simulink model "test_canards_sim"  (R2026b)
settings: Solver=VariableStepAuto  StopTime=25
values from neighbouring files (symbols this model uses):
  Area = 0.014    [Full_Rocket_Constants.m]    (also in TestRocketSetup.m = 0.00817128249199)
  BF_H = 0.14    [Full_Rocket_Constants.m]    (also in TestRocketSetup.m = 0.102)
  BF_NFins = 4    [Full_Rocket_Constants.m]    (also in TestRocketSetup.m)
  BF_plan = ((BF_TC+BF_RC)/2)*BF_H    (= 0.0329)    [Full_Rocket_Constants.m]    (also in TestRocketSetup.m = 0.0162129)
  BF_SA = deg2rad(58.3)    [Full_Rocket_Constants.m]    (also in TestRocketSetup.m = atan(BF_SL/BF_H))
  BF_t = 0.003    [TestRocketSetup.m]
  BF_X = 7.00    (= 7)    [Full_Rocket_Constants.m]    (also in TestRocketSetup.m = 1.626)
  BF_yMac = (BF_H/3)*((BF_RC+(2*BF_TC))/(BF_RC+BF_TC))    (= 0.0617588652482)    [Full_Rocket_Constants.m]    (also in TestRocketSetup.m = 0.0435080213904)
  boost_end = boosterCurve(length(boosterCurve), 1)    [Full_Rocket_Constants.m]    (also in TestRocketSetup.m)
  boost_start = boosterCurve(1, 1)    [Full_Rocket_Constants.m]    (also in TestRocketSetup.m)
  boost_t_cg = boost_data(:,1)    [Full_Rocket_Constants.m]    (also in TestRocketSetup.m)
  boost_x_cg = boost_data(:,3)    [Full_Rocket_Constants.m]    (also in TestRocketSetup.m = boost_data(:,3)/100)
  Booster_Length = 4.73    [Full_Rocket_Constants.m]    (also in TestRocketSetup.m = 1.92)
  Booster_MotorDiam = 0.098    [Full_Rocket_Constants.m]    (also in TestRocketSetup.m = 0.075)
  boosterCurve = thrustCurve("Data/Cesaroni_2856L910-P.csv")    [TestRocketSetup.m]
  boosterISP = 223    [Full_Rocket_Constants.m]    (also in TestRocketSetup.m = 229)
  cbar_BF = (2/3)*(BF_RC^2 + BF_RC*BF_TC + BF_TC^2)/(BF_RC + BF_TC)    (= 0.244771631206)    [Full_Rocket_Constants.m]    (also in TestRocketSetup.m = 0.169240452973)
  cbar_CR = CR_Plan/CR_Span    [Full_Rocket_Constants.m]    (also in TestRocketSetup.m = 0.0169333333333)
  CR_LE = atan(CR_SL/CR_Span)    [TestRocketSetup.m]
  CR_mC = 0    [Full_Rocket_Constants.m]    (also in TestRocketSetup.m = atan((CR_SL + CR_TC/2 - CR_RC/2)/CR_Span))
  CR_Plan = 0    [Full_Rocket_Constants.m]    (also in TestRocketSetup.m = 0.000381)
  CR_pos = 0    [Full_Rocket_Constants.m]    (also in TestRocketSetup.m = 0.495166666667)
  CR_Span = sqrt(CR_AR*CR_Plan)    [Full_Rocket_Constants.m]    (also in TestRocketSetup.m = 0.03)
  CR_t = 0.003    [TestRocketSetup.m]
  CR_yMAC = (CR_Span/3)*(CR_RC + 2*CR_TC)/(CR_RC + CR_TC)    (= 0.01)    [TestRocketSetup.m]
  Diam = 0.157    [Full_Rocket_Constants.m]    (also in TestRocketSetup.m = 0.102)
  Gc_BF = atan((BF_SL + BF_TC/2 - BF_RC/2)/BF_H)    [Full_Rocket_Constants.m]    (also in TestRocketSetup.m)
  Ixx_empty = 0.016109    [TestRocketSetup.m]
  Ixx_full = 0.017068    [TestRocketSetup.m]
  Iyy_empty = 3.018769    [TestRocketSetup.m]
  Iyy_full = 3.518905    [TestRocketSetup.m]
  NC_aBase = pi*(NC_dBase/2)^2    (= 0.0134782178821)    [Full_Rocket_Constants.m]    (also in TestRocketSetup.m = 0.00817128249199)
  NC_aPlan = 0.03355206    [Full_Rocket_Constants.m]    (also in TestRocketSetup.m = integral(@(x) 2*NC_rx(x), 0, NC_L))
  NC_aTop = pi*(NC_dTop/2)^2    (= 0)    [Full_Rocket_Constants.m]    (also in TestRocketSetup.m = 7.85398163397e-19)
  NC_CP = NC_L*0.466    (= 0.177546)    [Full_Rocket_Constants.m]    (also in TestRocketSetup.m = 0.189196)
  NC_dBase = 0.131    [Full_Rocket_Constants.m]    (also in TestRocketSetup.m = 0.102)
  NC_kappa = 1    [TestRocketSetup.m]
  NC_L = 0.381    [Full_Rocket_Constants.m]    (also in TestRocketSetup.m = 0.406)
  NC_phiJoint = 0    [TestRocketSetup.m]
  NC_Xlift = NC_Xlift_numerator / NC_aPlan    [Full_Rocket_Constants.m]    (also in TestRocketSetup.m)
  SC_L =     [Full_Rocket_Constants.m]    (also in TestRocketSetup.m = 0.229)
  spincan_radius = 0.0889    [Full_Rocket_Constants.m]    (also in TestRocketSetup.m = 0.0635)
  SurfaceRoughness = 60e-6    (= 6e-05)    [Full_Rocket_Constants.m]    (also in TestRocketSetup.m)
  TR_L =     [Full_Rocket_Constants.m]    (also in TestRocketSetup.m = 0.102)
  xMAC_BF = (BF_SL/3)*(BF_RC + 2*BF_TC)/(BF_RC + BF_TC)    (= 0.100137588652)    [Full_Rocket_Constants.m]    (also in TestRocketSetup.m = 0.0789116074237)
libraries: simulink x4, slpidlib x2, sl_discontinuities x2, aerolibwind2 x2, aerolibanim x1, aerolibatmos2 x1, aerolibasang x1
settings Model: SimulationMode=accelerator  Creator=linda  LastModifiedBy=linda
settings RTWCC: GPUComputeCapability=5.0

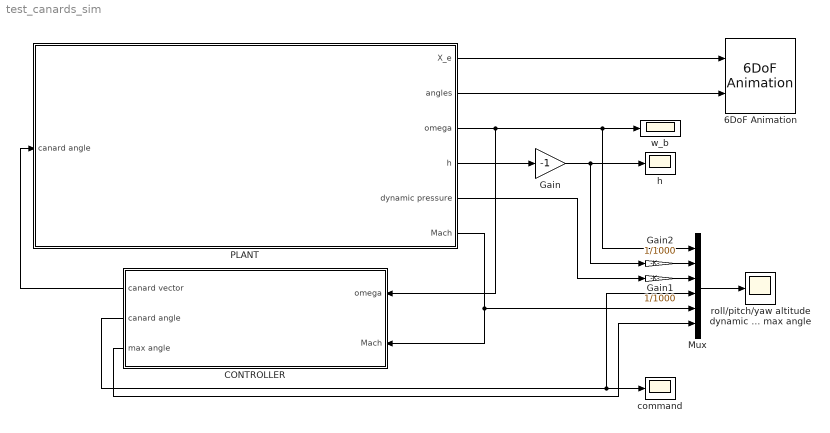
== system test_canards_sim ==
  6DoF Animation : aerolibanim/6DoF Animation  u1=[-1000 1000 -1000 1000 -2500 100]  u2=0.1  u3=250  u4=[1e6 1e6 1e6]  u5=Fixed position  u6=[3000 -3200 -1200]  u7=35  u8=on
  CONTROLLER : Subsystem
      settings: PortSchema="{\"entries\":[{\"content\":{\"sides\":[{\"content\":{\"connectorIds\":[\"Out1\",\"Out2\",\"Out3\"]},\"type\":\"ConnectorPlacement.EquallySpacedRectSide\",\"uuid\":\"acb4eb02-5623-4936-ab90-b0a31d594ccc\"},{\"content\":{\"connectorIds\":[\"In1\",\"In2\"],\"side\":\"RIGHT\"},\"type\":\"ConnectorPlacement.EquallySpacedRectSide\",\"uuid\":\"32f7e7ec-6d55-4d58-a621-02218861ecad\"},{\"content\":{\"side\":\"TOP\"},\"type\":\"ConnectorPlacement.EquallySpacedRectSide\",\"uuid\":\"63922e56-f870-4494-8f72-8c2e527eb7e4\"}]},\"type\":\"ConnectorPlacement.EquallySpacedConnector\",\"uuid\":\"1a722234-757d-46dd-a7b9-af51da458303\"}],\"packageUris\":[\"http://schema.mathworks.com/mf0/Connector/R2020b\"],\"version\":\"1.0\"}"
  Gain : Gain  Gain=-1
  Gain1 : Gain  Gain=1/1000
  Gain2 : Gain  Gain=1/1000
  Mux : Mux  Inputs=6
  PLANT : Subsystem
  command : Scope
      settings: ActiveDisplayYMinimum=-0.098392544287147957  ActiveDisplayYMaximum=0.020869012493307838  DataLoggingVariableName=ScopeData3
  h : Scope
      settings: ActiveDisplayYMinimum=1452.8796933312713  ActiveDisplayYMaximum=2766.4256793789323  DataLoggingVariableName=ScopeData2
  roll/pitch/yaw altitude dynamic pressure command mach max angle : Scope
      settings: ActiveDisplayYMinimum=-0.92690613477267036  ActiveDisplayYMaximum=0.910025444475978  DataLoggingVariableName=ScopeData4
  w_b : Scope
      settings: ActiveDisplayYMinimum=-3.5754328935781414  ActiveDisplayYMaximum=12.108972824331008
  wires:
  CONTROLLER/1(canard vector) -> PLANT/1(canard angle)
  PLANT/1(X_e) -> 6DoF Animation/1
  PLANT/2(angles) -> 6DoF Animation/2
  PLANT/3(omega) -> Mux/1, w_b/1, CONTROLLER/1(omega)
  PLANT/4(h) -> Gain/1
  Gain/1 -> Gain2/1, h/1
  CONTROLLER/2(canard angle) -> command/1, Mux/4
  Mux/1 -> roll/pitch/yaw altitude dynamic pressure command mach max angle/1
  Gain1/1 -> Mux/3
  PLANT/5(dynamic pressure) -> Gain1/1
  Gain2/1 -> Mux/2
  PLANT/6(Mach) -> CONTROLLER/2(Mach), Mux/5
  CONTROLLER/3(max angle) -> Mux/6

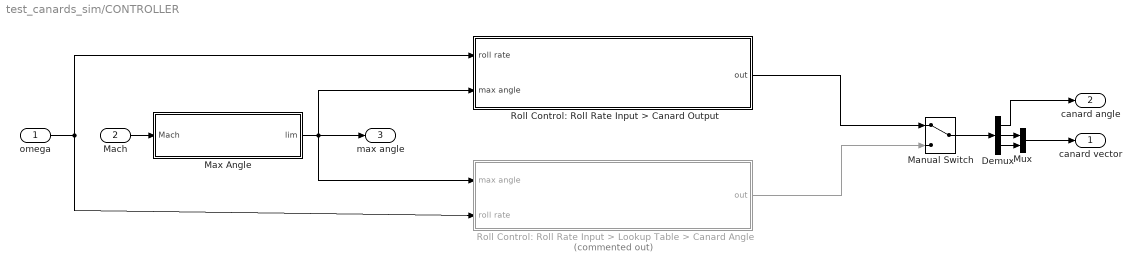
== system test_canards_sim/CONTROLLER ==
  omega : Inport
  Mach : Inport  Port=2
  Demux : Demux  Outputs=3
  Manual Switch : ManualSwitch
  Max Angle : Subsystem
  Mux : Mux  Inputs=2
  Roll Control: Roll Rate Input > Canard Output : Subsystem
  Roll Control: Roll Rate Input > Lookup Table > Canard Angle : Subsystem  Commented=on
  canard vector : Outport
  canard angle : Outport  Port=2
  max angle : Outport  Port=3
  wires:
  omega/1 -> Roll Control: Roll Rate Input > Canard Output/1(roll rate), Roll Control: Roll Rate Input > Lookup Table > Canard Angle/2(roll rate)
  Mach/1 -> Max Angle/1(Mach)
  Max Angle/1(lim) -> Roll Control: Roll Rate Input > Lookup Table > Canard Angle/1(max angle), Roll Control: Roll Rate Input > Canard Output/2(max angle), max angle/1
  Roll Control: Roll Rate Input > Canard Output/1(out) -> Manual Switch/1
  Manual Switch/1 -> Demux/1
  Demux/1 -> canard angle/1
  Roll Control: Roll Rate Input > Lookup Table > Canard Angle/1(out) -> Manual Switch/2
  Demux/2 -> Mux/1
  Demux/3 -> Mux/2
  Mux/1 -> canard vector/1

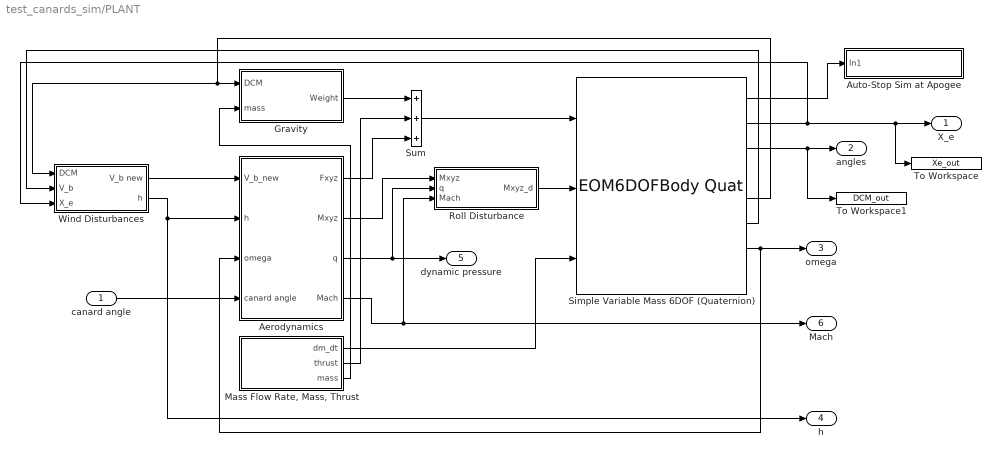
== system test_canards_sim/PLANT ==
  canard angle : Inport
  Aerodynamics : Subsystem
  Auto-Stop Sim at Apogee : Subsystem
  Gravity : Subsystem
  "Mass Flow Rate, Mass, Thrust" : Subsystem
  Roll Disturbance : Subsystem
  Simple Variable Mass 6DOF (Quaternion) : EOM6DOFBodyQuat  mtype=Simple Variable  eul_0=[0 deg2rad(85) 0]  mass_0=BoosterWetMass  mass_e=BoosterBurnoutMass  mass_f=BoosterWetMass  inertia_e=diag([Ixx_empty, Iyy_empty, Iyy_empty])  inertia_f=diag([Ixx_full, Iyy_full, Iyy_full])
  Sum : Sum  Inputs=+++
  To Workspace : ToWorkspace  VariableName=Xe_out  SaveFormat=Timeseries  SampleTime=-1
  To Workspace1 : ToWorkspace  VariableName=DCM_out  SaveFormat=Timeseries  SampleTime=-1
  Wind Disturbances : Subsystem
  X_e : Outport
  angles : Outport  Port=2
  omega : Outport  Port=3
  h : Outport  Port=4
  dynamic pressure : Outport  Port=5
  Mach : Outport  Port=6
  wires:
  Wind Disturbances/2(h) -> h/1, Aerodynamics/2(h)
  Simple Variable Mass 6DOF (Quaternion)/7 -> omega/1, Aerodynamics/3(omega)
  Simple Variable Mass 6DOF (Quaternion)/2 -> To Workspace/1, X_e/1, Wind Disturbances/3(X_e)
  Sum/1 -> Simple Variable Mass 6DOF (Quaternion)/1
  Gravity/1(Weight) -> Sum/1
  Aerodynamics/1(Fxyz) -> Sum/3
  Simple Variable Mass 6DOF (Quaternion)/5 -> Wind Disturbances/1(DCM), Gravity/1(DCM)
  Wind Disturbances/1(V_b new) -> Aerodynamics/1(V_b_new)
  Simple Variable Mass 6DOF (Quaternion)/6 -> Wind Disturbances/2(V_b)
  "Mass Flow Rate, Mass, Thrust"/1(dm_dt) -> Simple Variable Mass 6DOF (Quaternion)/3
  "Mass Flow Rate, Mass, Thrust"/2(thrust) -> Sum/2
  "Mass Flow Rate, Mass, Thrust"/3(mass) -> Gravity/2(mass)
  Simple Variable Mass 6DOF (Quaternion)/1 -> Auto-Stop Sim at Apogee/1(In1)
  Simple Variable Mass 6DOF (Quaternion)/3 -> To Workspace1/1, angles/1
  canard angle/1 -> Aerodynamics/4(canard angle)
  Aerodynamics/2(Mxyz) -> Roll Disturbance/1(Mxyz)
  Roll Disturbance/1(Mxyz_d) -> Simple Variable Mass 6DOF (Quaternion)/2
  Aerodynamics/3(q) -> dynamic pressure/1, Roll Disturbance/2(q)
  Aerodynamics/4(Mach) -> Roll Disturbance/3(Mach), Mach/1

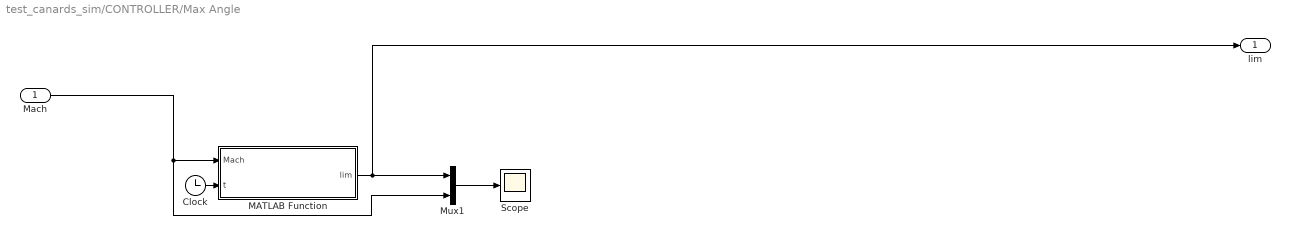
== system test_canards_sim/CONTROLLER/Max Angle ==
  Mach : Inport
  Clock : Clock
  MATLAB Function : MATLAB Function  TreatAsAtomicUnit=on
  Mux1 : Mux  Inputs=2
  Scope : Scope
      settings: ActiveDisplayYMinimum=-0.10058311536277464  ActiveDisplayYMaximum=0.91689608071086814  DataLoggingVariableName=ScopeData8
  lim : Outport
  wires:
  Clock/1 -> MATLAB Function/2(t)
  Mach/1 -> MATLAB Function/1(Mach), Mux1/2
  MATLAB Function/1(lim) -> lim/1, Mux1/1
  Mux1/1 -> Scope/1

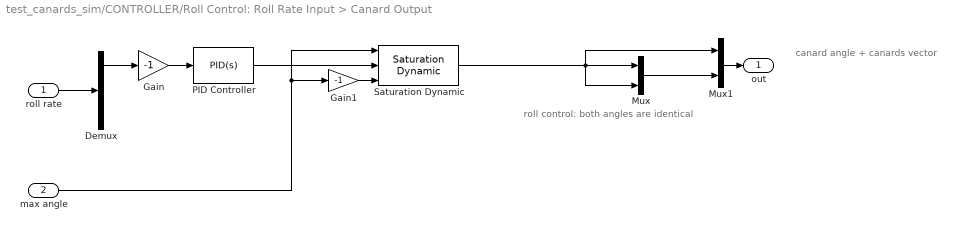
== system test_canards_sim/CONTROLLER/Roll Control: Roll Rate Input > Canard Output ==
  note: canard angle
      | +
      | canards vector
  note: roll control: both angles are identical
  roll rate : Inport
  max angle : Inport  Port=2
  Demux : Demux  Outputs=3
  Gain : Gain  Gain=-1
  Gain1 : Gain  Gain=-1
  Mux : Mux  Inputs=2
  Mux1 : Mux  Inputs=2
  PID Controller : slpidlib/PID Controller  Controller=PID  Form=Parallel  TimeDomain=Continuous-time  UseExternalTs=off  SampleTime=-1  IntegratorMethod=Forward Euler  FilterMethod=Forward Euler  ControllerParametersSource=internal  P=2.1  I=0.75  UseKiTs=off  D=0.2  UseExternalDerivativeSource=off  N=100  UseFilter=on  TunerSelectOption=Transfer Function Based (PID Tuner App)  InitialConditionSource=internal  InitialConditionForIntegrator=0  InitialConditionForFilter=0  DifferentiatorICPrevScaledInput=0  ExternalReset=none  TrackingMode=off  Kt=1  LimitOutput=off  SatLimitsSource=internal  UpperSaturationLimit=deg2rad(15)  LowerSaturationLimit=deg2rad(-15)  LinearizeAsGain=on  AntiWindupMode=clamping  Kb=1  LimitIntegrator=off  UpperIntegratorSaturationLimit=inf  LowerIntegratorSaturationLimit=-inf  POutMin=[]  POutMax=[]  IOutMin=[]  IOutMax=[]  DOutMin=[]  DOutMax=[]  NOutMin=[]  NOutMax=[]  SumOutMin=[]  SumOutMax=[]  SaturationOutMin=[]  SaturationOutMax=[]  PParamMin=[]  PParamMax=[]  IParamMin=[]  IParamMax=[]  DParamMin=[]  DParamMax=[]  NParamMin=[]  NParamMax=[]  KbParamMin=[]  KbParamMax=[]  KtParamMin=[]  KtParamMax=[]  KbOutMin=[]  KbOutMax=[]  KtOutMin=[]  KtOutMax=[]  IntegratorOutMin=[]  IntegratorOutMax=[]  FilterOutMin=[]  FilterOutMax=[]  SumI1OutMin=[]  SumI1OutMax=[]  SumI2OutMin=[]  SumI2OutMax=[]  SumI3OutMin=[]  SumI3OutMax=[]  SumI4OutMin=[]  SumI4OutMax=[]  SumDOutMin=[]  SumDOutMax=[]  DifferentiatorOutMin=[]  DifferentiatorOutMax=[]  FilterDiffOutCoefMin=[]  FilterDiffOutCoefMax=[]  ReciprocalOutMin=[]  ReciprocalOutMax=[]  SumDenOutMin=[]  SumDenOutMax=[]  SumNumOutMin=[]  SumNumOutMax=[]  DivideOutMin=[]  DivideOutMax=[]  UdiffTsProdOutMin=[]  UdiffTsProdOutMax=[]  NTsProdOutMin=[]  NTsProdOutMax=[]  UintegralTsProdOutMin=[]  UintegralTsProdOutMax=[]  UngainTsProdOutMin=[]  UngainTsProdOutMax=[]  ClampingZeroOutDataTypeStr=Inherit: Inherit via back propagation  ClampingZeroOutMin=[]  ClampingZeroOutMax=[]  FilterDenConstantOutDataTypeStr=Inherit: Inherit via back propagation  FilterDenConstantOutMin=[]  FilterDenConstantOutMax=[]  PCopyOutDataTypeStr=Inherit: Inherit via back propagation  PCopyOutMin=[]  PCopyOutMax=[]  NCopyOutDataTypeStr=Inherit: Inherit via back propagation  NCopyOutMin=[]  NCopyOutMax=[]  IntegratorContinuousStateAttributes=''  IntegratorStateMustResolveToSignalObject=off  IntegratorRTWStateStorageClass=Auto  FilterContinuousStateAttributes=''  FilterStateMustResolveToSignalObject=off  FilterRTWStateStorageClass=Auto  ParallelPVariant=InternalParameters  IdealPVariant=Disabled  IVariant=InternalParameters  DVariant=InternalParameters  IntegratorVariant=Continuous  SatVariant=Disabled  AWVariant=Passthrough  PCopyVariant=Disabled  TRVariant=Disabled  FdbkBlocksVariant=Forward  IdealPFdbkVariant=Disabled  SatFdbkVariant=Disabled  DerivativeFilterVariant=ContFilter  NVariant=InternalParameters  NCopyVariant=Disabled  FilterICVariant=InternalICsFilter  IntegratorICVariant=InternalICs  ExternalResetVariant=Disabled  TRSumVariant=Passthrough  SumFdbkVariant=Disabled  SumVariant=Sum_PID  TsampFilterVariant=InternalTs  TsampNgainVariant=Passthrough  TsampIntegralVariant=Disabled_SignalSpec  ExternalSaturationOutDataTypeStr=Inherit: Same as second input  DerivativeSourceVariant=ErrorSignal  PreIntVariant=InternalPreInt
  Saturation Dynamic : sl_discontinuities/Saturation Dynamic  OutMin=[]  OutMax=[]  OutDataTypeStr=Inherit: Same as second input  OutDataType=fixdt(1, 16)  OutScaling=2^-10  DoSatur=off
      settings: LibrarySourceBlock=|
      | simulink/Discontinuities/Saturation
      | Dynamic
  out : Outport
  wires:
  Demux/1 -> Gain/1
  Gain/1 -> PID Controller/1
  Gain1/1 -> Saturation Dynamic/3
  PID Controller/1 -> Saturation Dynamic/2
  Saturation Dynamic/1 -> Mux1/1, Mux/2, Mux/1
  Mux/1 -> Mux1/2
  roll rate/1 -> Demux/1
  max angle/1 -> Gain1/1, Saturation Dynamic/1
  Mux1/1 -> out/1

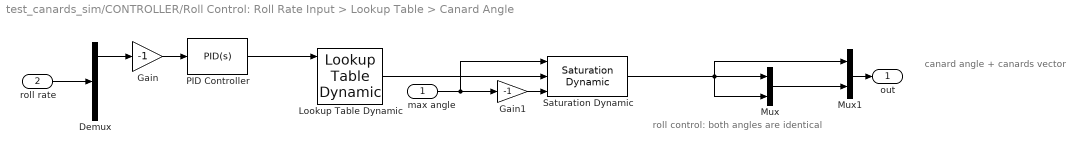
== system test_canards_sim/CONTROLLER/Roll Control: Roll Rate Input > Lookup Table > Canard Angle ==
  note: canard angle
      | +
      | canards vector
  note: roll control: both angles are identical
  max angle : Inport
  roll rate : Inport  Port=2
  Demux : Demux  Outputs=3
  Gain : Gain  Gain=-1
  Gain1 : Gain  Gain=-1
  Lookup Table Dynamic : simulink/Lookup Tables/Lookup Table Dynamic  LookUpMeth=Interpolation-Use End Values  OutDataType=fixdt('double')  OutScaling=2^-10  OutputDataTypeScalingMode=Specify via dialog  OutDataTypeStr=double  DoSatur=off
  Mux : Mux  Inputs=2
  Mux1 : Mux  Inputs=2
  PID Controller : slpidlib/PID Controller  Controller=PID  Form=Parallel  TimeDomain=Continuous-time  UseExternalTs=off  SampleTime=-1  IntegratorMethod=Forward Euler  FilterMethod=Forward Euler  ControllerParametersSource=internal  P=2.1  I=0.75  UseKiTs=off  D=0.2  UseExternalDerivativeSource=off  N=100  UseFilter=on  TunerSelectOption=Transfer Function Based (PID Tuner App)  InitialConditionSource=internal  InitialConditionForIntegrator=0  InitialConditionForFilter=0  DifferentiatorICPrevScaledInput=0  ExternalReset=none  TrackingMode=off  Kt=1  LimitOutput=off  SatLimitsSource=internal  UpperSaturationLimit=deg2rad(15)  LowerSaturationLimit=deg2rad(-15)  LinearizeAsGain=on  AntiWindupMode=clamping  Kb=1  LimitIntegrator=off  UpperIntegratorSaturationLimit=inf  LowerIntegratorSaturationLimit=-inf  POutMin=[]  POutMax=[]  IOutMin=[]  IOutMax=[]  DOutMin=[]  DOutMax=[]  NOutMin=[]  NOutMax=[]  SumOutMin=[]  SumOutMax=[]  SaturationOutMin=[]  SaturationOutMax=[]  PParamMin=[]  PParamMax=[]  IParamMin=[]  IParamMax=[]  DParamMin=[]  DParamMax=[]  NParamMin=[]  NParamMax=[]  KbParamMin=[]  KbParamMax=[]  KtParamMin=[]  KtParamMax=[]  KbOutMin=[]  KbOutMax=[]  KtOutMin=[]  KtOutMax=[]  IntegratorOutMin=[]  IntegratorOutMax=[]  FilterOutMin=[]  FilterOutMax=[]  SumI1OutMin=[]  SumI1OutMax=[]  SumI2OutMin=[]  SumI2OutMax=[]  SumI3OutMin=[]  SumI3OutMax=[]  SumI4OutMin=[]  SumI4OutMax=[]  SumDOutMin=[]  SumDOutMax=[]  DifferentiatorOutMin=[]  DifferentiatorOutMax=[]  FilterDiffOutCoefMin=[]  FilterDiffOutCoefMax=[]  ReciprocalOutMin=[]  ReciprocalOutMax=[]  SumDenOutMin=[]  SumDenOutMax=[]  SumNumOutMin=[]  SumNumOutMax=[]  DivideOutMin=[]  DivideOutMax=[]  UdiffTsProdOutMin=[]  UdiffTsProdOutMax=[]  NTsProdOutMin=[]  NTsProdOutMax=[]  UintegralTsProdOutMin=[]  UintegralTsProdOutMax=[]  UngainTsProdOutMin=[]  UngainTsProdOutMax=[]  ClampingZeroOutDataTypeStr=Inherit: Inherit via back propagation  ClampingZeroOutMin=[]  ClampingZeroOutMax=[]  FilterDenConstantOutDataTypeStr=Inherit: Inherit via back propagation  FilterDenConstantOutMin=[]  FilterDenConstantOutMax=[]  PCopyOutDataTypeStr=Inherit: Inherit via back propagation  PCopyOutMin=[]  PCopyOutMax=[]  NCopyOutDataTypeStr=Inherit: Inherit via back propagation  NCopyOutMin=[]  NCopyOutMax=[]  IntegratorContinuousStateAttributes=''  IntegratorStateMustResolveToSignalObject=off  IntegratorRTWStateStorageClass=Auto  FilterContinuousStateAttributes=''  FilterStateMustResolveToSignalObject=off  FilterRTWStateStorageClass=Auto  ParallelPVariant=InternalParameters  IdealPVariant=Disabled  IVariant=InternalParameters  DVariant=InternalParameters  IntegratorVariant=Continuous  SatVariant=Disabled  AWVariant=Passthrough  PCopyVariant=Disabled  TRVariant=Disabled  FdbkBlocksVariant=Forward  IdealPFdbkVariant=Disabled  SatFdbkVariant=Disabled  DerivativeFilterVariant=ContFilter  NVariant=InternalParameters  NCopyVariant=Disabled  FilterICVariant=InternalICsFilter  IntegratorICVariant=InternalICs  ExternalResetVariant=Disabled  TRSumVariant=Passthrough  SumFdbkVariant=Disabled  SumVariant=Sum_PID  TsampFilterVariant=InternalTs  TsampNgainVariant=Passthrough  TsampIntegralVariant=Disabled_SignalSpec  ExternalSaturationOutDataTypeStr=Inherit: Same as second input  DerivativeSourceVariant=ErrorSignal  PreIntVariant=InternalPreInt
  Saturation Dynamic : sl_discontinuities/Saturation Dynamic  OutMin=[]  OutMax=[]  OutDataTypeStr=Inherit: Same as second input  OutDataType=fixdt(1, 16)  OutScaling=2^-10  DoSatur=off
      settings: LibrarySourceBlock=|
      | simulink/Discontinuities/Saturation
      | Dynamic
  out : Outport
  wires:
  Gain/1 -> PID Controller/1
  Demux/1 -> Gain/1
  Gain1/1 -> Saturation Dynamic/3
  roll rate/1 -> Demux/1
  max angle/1 -> Gain1/1, Saturation Dynamic/1
  Mux/1 -> Mux1/2
  Mux1/1 -> out/1
  Saturation Dynamic/1 -> Mux1/1, Mux/2, Mux/1
  PID Controller/1 -> Lookup Table Dynamic/1
  Lookup Table Dynamic/1 -> Saturation Dynamic/2

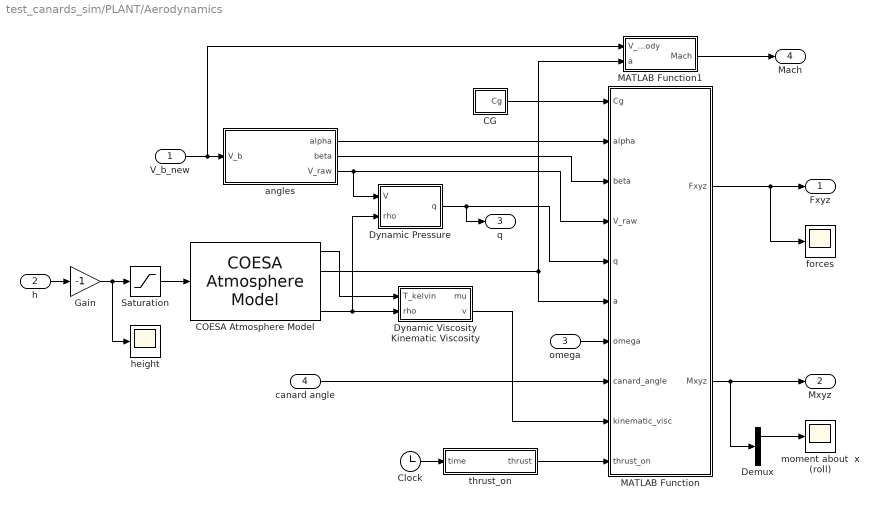
== system test_canards_sim/PLANT/Aerodynamics ==
  V_b_new : Inport
  h : Inport  Port=2
  omega : Inport  Port=3
  canard angle : Inport  Port=4
  " thrust_on" : MATLAB Function  TreatAsAtomicUnit=on
  CG : Subsystem
  COESA Atmosphere Model : aerolibatmos2/COESA Atmosphere Model  units=Metric (MKS)  spec=1976 COESA-extended U.S. Standard Atmosphere  model=Profile  profile_var=High temperature  profile_percent=1%  profile_alt=5 km (16404 ft)  envelope_var=High temperature  envelope_percent=1%  action=Warning
  Clock : Clock
  Demux : Demux  Outputs=3
  Dynamic Pressure : MATLAB Function  TreatAsAtomicUnit=on
  Dynamic Viscosity Kinematic Viscosity : MATLAB Function  TreatAsAtomicUnit=on
  Gain : Gain  Gain=-1
  MATLAB Function : MATLAB Function  TreatAsAtomicUnit=on
  MATLAB Function1 : MATLAB Function  TreatAsAtomicUnit=on
  Saturation : Saturate  UpperLimit=84852  LowerLimit=0
  angles : MATLAB Function  TreatAsAtomicUnit=on
  forces : Scope
      settings: ActiveDisplayYMinimum=-21.307515868467224  ActiveDisplayYMaximum=16.150178192243292
  height : Scope
      settings: ActiveDisplayYMinimum=-4.5744937595802373  ActiveDisplayYMaximum=46.098202210324679  DataLoggingVariableName=ScopeData5
  moment about  x (roll) : Scope
      settings: ActiveDisplayYMinimum=-28.928384383300997  ActiveDisplayYMaximum=28.04821872272084  DataLoggingVariableName=ScopeData6
  Fxyz : Outport
  Mxyz : Outport  Port=2
  q : Outport  Port=3
  Mach : Outport  Port=4
  wires:
  COESA Atmosphere Model/1 -> Dynamic Viscosity Kinematic Viscosity/1(T_kelvin)
  COESA Atmosphere Model/4 -> Dynamic Viscosity Kinematic Viscosity/2(rho), Dynamic Pressure/2(rho)
  Dynamic Viscosity Kinematic Viscosity/2(v) -> MATLAB Function/9(kinematic_visc)
  Dynamic Pressure/1(q) -> MATLAB Function/5(q), q/1
  COESA Atmosphere Model/2 -> MATLAB Function/6(a), MATLAB Function1/2(a)
  MATLAB Function/1(Fxyz) -> forces/1, Fxyz/1
  MATLAB Function/2(Mxyz) -> Mxyz/1, Demux/1
  " thrust_on"/1(thrust) -> MATLAB Function/10(thrust_on)
  omega/1 -> MATLAB Function/7(omega)
  CG/1(Cg) -> MATLAB Function/1(Cg)
  canard angle/1 -> MATLAB Function/8(canard_angle)
  V_b_new/1 -> angles/1(V_b), MATLAB Function1/1(V_air_body)
  angles/3(V_raw) -> MATLAB Function/4(V_raw), Dynamic Pressure/1(V)
  angles/2(beta) -> MATLAB Function/3(beta)
  angles/1(alpha) -> MATLAB Function/2(alpha)
  Clock/1 -> " thrust_on"/1(time)
  h/1 -> Gain/1
  Gain/1 -> height/1, Saturation/1
  Saturation/1 -> COESA Atmosphere Model/1
  Demux/1 -> moment about  x (roll)/1
  MATLAB Function1/1(Mach) -> Mach/1

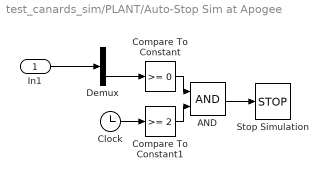
== system test_canards_sim/PLANT/Auto-Stop Sim at Apogee ==
  In1 : Inport
  AND : Logic  IconShape=distinctive  AllPortsSameDT=off  OutDataTypeStr=boolean
  Clock : Clock
  Compare To Constant : simulink/Logic and Bit Operations/Compare To Constant  relop=>=  const=0  OutDataTypeStr=boolean
  Compare To Constant1 : simulink/Logic and Bit Operations/Compare To Constant  relop=>=  const=2  OutDataTypeStr=boolean
  Demux : Demux  Outputs=3
  Stop Simulation : Stop
  wires:
  Demux/3 -> Compare To Constant/1
  Compare To Constant/1 -> AND/1
  AND/1 -> Stop Simulation/1
  Clock/1 -> Compare To Constant1/1
  In1/1 -> Demux/1
  Compare To Constant1/1 -> AND/2

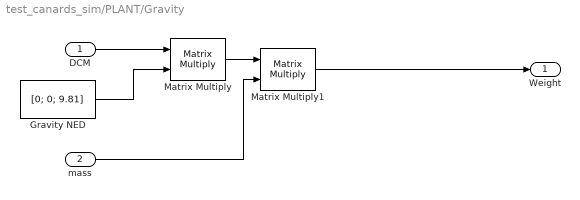
== system test_canards_sim/PLANT/Gravity ==
  DCM : Inport
  mass : Inport  Port=2
  Gravity NED : Constant  Value=[0; 0; 9.81]
  Matrix Multiply : Product  Multiplication=Matrix(*)
  Matrix Multiply1 : Product  Multiplication=Matrix(*)
  Weight : Outport
  wires:
  DCM/1 -> Matrix Multiply/1
  Gravity NED/1 -> Matrix Multiply/2
  Matrix Multiply1/1 -> Weight/1
  mass/1 -> Matrix Multiply1/2
  Matrix Multiply/1 -> Matrix Multiply1/1

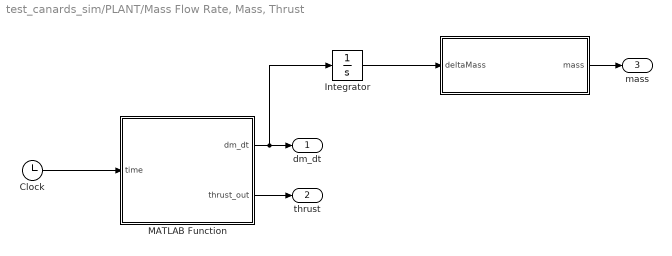
== system test_canards_sim/PLANT/Mass Flow Rate, Mass, Thrust ==
  " " : MATLAB Function  TreatAsAtomicUnit=on
  Clock : Clock
  Integrator : Integrator
  MATLAB Function : MATLAB Function  TreatAsAtomicUnit=on
  dm_dt : Outport
  thrust : Outport  Port=2
  mass : Outport  Port=3
  wires:
  Clock/1 -> MATLAB Function/1(time)
  MATLAB Function/1(dm_dt) -> Integrator/1, dm_dt/1
  MATLAB Function/2(thrust_out) -> thrust/1
  Integrator/1 -> " "/1(deltaMass)
  " "/1(mass) -> mass/1

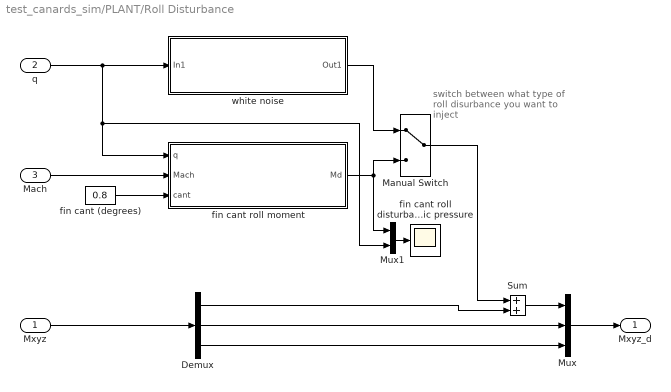
== system test_canards_sim/PLANT/Roll Disturbance ==
  note: switch between
      | what type of roll
      | disurbance you
      | want to inject
  Mxyz : Inport
  q : Inport  Port=2
  Mach : Inport  Port=3
  Demux : Demux  Outputs=3
  Manual Switch : ManualSwitch
  Mux : Mux  Inputs=3
  Mux1 : Mux  Inputs=2
  Sum : Sum
  fin cant (degrees) : Constant  Value=0.8
  fin cant roll disturbance & dynamic pressure : Scope
      settings: ActiveDisplayYMinimum=-1.1548840832620328  ActiveDisplayYMaximum=10.497326561375871  DataLoggingVariableName=ScopeData7
  fin cant roll moment : MATLAB Function  TreatAsAtomicUnit=on
  white noise : Subsystem
  Mxyz_d : Outport
  wires:
  Sum/1 -> Mux/1
  Demux/3 -> Mux/3
  Demux/2 -> Mux/2
  Demux/1 -> Sum/2
  q/1 -> Mux1/2, fin cant roll moment/1(q), white noise/1(In1)
  Mxyz/1 -> Demux/1
  Mux/1 -> Mxyz_d/1
  white noise/1(Out1) -> Manual Switch/1
  Manual Switch/1 -> Sum/1
  fin cant roll moment/1(Md) -> Mux1/1, Manual Switch/2
  Mach/1 -> fin cant roll moment/2(Mach)
  fin cant (degrees)/1 -> fin cant roll moment/3(cant)
  Mux1/1 -> fin cant roll disturbance & dynamic pressure/1

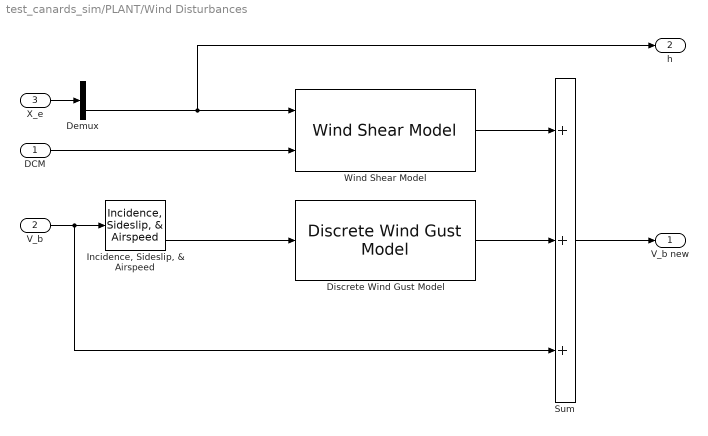
== system test_canards_sim/PLANT/Wind Disturbances ==
  DCM : Inport
  V_b : Inport  Port=2
  X_e : Inport  Port=3
  Demux : Demux  Outputs=3
  Discrete Wind Gust Model : aerolibwind2/Discrete Wind Gust Model  units=Metric (MKS)  Gx=on  Gy=on  Gz=on  t_0=5  d_m=[120 120 80]  v_m=[3.5 3.5 3.0]
  "Incidence, Sideslip, & Airspeed" : aerolibasang/Incidence, Sideslip, & Airspeed
  Sum : Sum  Inputs=+++
  Wind Shear Model : aerolibwind2/Wind Shear Model  units=Metric (MKS)  phase=Category C - Terminal Flight Phase  W_20=15  Wdeg=30
  V_b new : Outport
  h : Outport  Port=2
  wires:
  V_b/1 -> Sum/3, "Incidence, Sideslip, & Airspeed"/1
  "Incidence, Sideslip, & Airspeed"/3 -> Discrete Wind Gust Model/1
  Wind Shear Model/1 -> Sum/1
  Discrete Wind Gust Model/1 -> Sum/2
  Sum/1 -> V_b new/1
  DCM/1 -> Wind Shear Model/2
  X_e/1 -> Demux/1
  Demux/3 -> h/1, Wind Shear Model/1

== system test_canards_sim/PLANT/Aerodynamics/CG ==
  Clock : Clock
  cg lookup table : Lookup_n-D  NumberOfTableDimensions=1  BreakpointsForDimension1=boost_t_cg  Table=boost_x_cg  ExtrapMethod=Clip  InternalRulePriority=Speed  RndMeth=Simplest
  Cg : Outport
  wires:
  Clock/1 -> cg lookup table/1
  cg lookup table/1 -> Cg/1

== system test_canards_sim/PLANT/Roll Disturbance/white noise ==
  In1 : Inport
  Band-Limited White Noise : simulink/Sources/Band-Limited White Noise  Cov=[0.1]  Ts=0.1  seed=[23341]
  Gain : Gain  Gain=1e-5
  Product : Product
  Scope : Scope
      settings: ActiveDisplayYMinimum=-0.70382533129315117  ActiveDisplayYMaximum=0.99177758444579689  DataLoggingVariableName=ScopeData7
  Out1 : Outport
  wires:
  Product/1 -> Out1/1, Scope/1
  Band-Limited White Noise/1 -> Gain/1
  In1/1 -> Product/1
  Gain/1 -> Product/2

== matlab function test_canards_sim/PLANT/Aerodynamics/Dynamic Viscosity Kinematic Viscosity ==
  data: T_kelvin input; mu output; rho input; v output
function [mu, v] = fcn(T_kelvin, rho)

% Sutherland's Law

mu_ref = 1.716e-5;  % Pa*s
T_ref = 273.15;     % Kelvin
S = 110.4;          % Kelvin

C1 = (mu_ref*(T_ref+S))/(T_ref^(1.5));

mu = (C1*(T_kelvin^1.5))/(T_kelvin + S);

v = mu/rho;
;

== matlab function test_canards_sim/PLANT/Mass Flow Rate, Mass, Thrust/MATLAB Function ==
  data: dm_dt output; boosterCurve parameter; boosterISP parameter; time input; thrust_out output
function [dm_dt, thrust_out] = mass_flow_rate(boosterCurve, boosterISP, time)
g0 = 9.80665;
thrust = interp1(boosterCurve(:,1), boosterCurve(:,2), time, 'linear', 0);  % 0 outside the curve
dm_dt = -(thrust / (g0 * boosterISP));
thrust_out = [thrust; 0; 0];  % [Fx; Fy; Fz], N
end

== matlab function test_canards_sim/PLANT/Mass Flow Rate, Mass, Thrust/  ==
  data: deltaMass input; mass output; BoosterWetMass parameter
function mass = current_mass(deltaMass, BoosterWetMass)
mass = BoosterWetMass + deltaMass;   % deltaMass is the integral of dm_dt, so it goes negative during the burn
end

== matlab function test_canards_sim/PLANT/Aerodynamics/ thrust_on ==
  data: time input; thrust output; boost_start parameter; boost_end parameter
function thrust = thrust_on(time, boost_start, boost_end)

if (boost_start <= time) && (time <= boost_end)
    thrust = 1;
else
    thrust = 0;
end

== matlab function test_canards_sim/PLANT/Aerodynamics/Dynamic Pressure ==
  data: V input; q output; rho input
function q = fcn(V, rho)
q = 0.5*rho*V^2;

== matlab function test_canards_sim/PLANT/Aerodynamics/angles ==
  data: V_b input; alpha output; beta output; V_raw output
function [alpha, beta, V_raw] = angles(V_b)
% V_b: air-relative body velocity from disturbances [m/s]

u = V_b(1);
v = V_b(2);
w = V_b(3);

V_raw = sqrt(u*u + v*v + w*w);

if V_raw < 1e-3
    alpha = 0;
    beta  = 0;
else
    alpha = atan2(w, u);
    beta  = atan2(v, sqrt(u*u + w*w));
end

== matlab function test_canards_sim/CONTROLLER/Max Angle/MATLAB Function ==
  settings: updateMethod=DISCRETE
  data: Mach input; lim output; t input; boost_end parameter
function lim = max_deflection(Mach, t, boost_end)

if t < boost_end
    lim_deg = 10; % climbing to Mach peak
else
    lim_deg = min(10 + 50*max(0.8 - Mach, 0), 45); % +5 deg per 0.1 Mach below 0.8
end
lim = deg2rad(lim_deg);
end

== matlab function test_canards_sim/PLANT/Roll Disturbance/fin cant roll moment ==
  data: Md output; q input; Mach input; cant input; BF_NFins parameter; BF_H parameter; BF_plan parameter; spincan_radius parameter; Area parameter; BF_yMac parameter; Gc_BF parameter
function Md = finCant_roll(q, Mach, cant, BF_NFins, BF_H, BF_plan, spincan_radius, Area, BF_yMac, Gc_BF)
% steady roll moment from a fin cant angle (same fin-set formulas as the aero code block)

M_ = min(Mach, 0.9); % subsonic Diederich formula (rocket peaks near Mach 0.8)
beta_c = sqrt(1 - M_^2); % Eq. 3.13
CNa1 = 2*pi*(BF_H^2/Area)/(1 + sqrt(1 + (beta_c*BF_H^2/(BF_plan*cos(Gc_BF)))^2)); % Eq. 3.40 (one fin, per rad)
xi = BF_yMac + spincan_radius; % Distance from roll axis to fin MAC
Md = BF_NFins * q * Area * CNa1 * deg2rad(cant) * xi; % Eq. 3.66

end

== matlab function test_canards_sim/PLANT/Aerodynamics/MATLAB Function1 ==
  data: V_air_body input; Mach output; a input
function Mach = calculate_mach(V_air_body, a)

V_air = sqrt(V_air_body(1)^2 + V_air_body(2)^2 + V_air_body(3)^2);

Mach = V_air / a;

end

== matlab function test_canards_sim/PLANT/Aerodynamics/MATLAB Function ==
  data: Fxyz output; Cg input; alpha input; beta input; V_raw input; q input; a input; omega input; canard_angle input; Mxyz output; kinematic_visc input; thrust_on input; Diam parameter; Area parameter; spincan_radius parameter; Booster_Length parameter; NC_CP parameter; NC_Xlift parameter; BF_X parameter; BF_t parameter; CR_Plan parameter; Booster_MotorDiam parameter; CR_pos parameter; SC_L parameter; NC_aBase parameter; NC_aPlan parameter; TR_L parameter; BF_H parameter; xMAC_BF parameter; SurfaceRoughness parameter; cbar_BF parameter; BF_NFins parameter; CR_Span parameter; CR_yMAC parameter; NC_L parameter; NC_aTop parameter; BF_plan parameter; BF_SA parameter; CR_mC parameter; NC_dBase parameter; CR_t parameter; Gc_BF parameter; cbar_CR parameter; NC_phiJoint parameter; CR_LE parameter; NC_kappa parameter
function [Fxyz, Mxyz] = aerodynamics(Cg, alpha, beta, V_raw, q, a, omega, canard_angle, kinematic_visc, thrust_on, ...
    Diam, Area, spincan_radius, Booster_Length, NC_CP, NC_Xlift, BF_X, BF_t, CR_Plan, Booster_MotorDiam, CR_pos,...
    SC_L, NC_aBase, NC_aPlan, TR_L, BF_H, xMAC_BF, SurfaceRoughness, cbar_BF, BF_NFins, CR_Span, CR_yMAC, ...
    NC_L, NC_aTop, BF_plan, BF_SA, CR_mC, NC_dBase, CR_t, Gc_BF, cbar_CR, NC_phiJoint, CR_LE, NC_kappa)

% Openrocket Documentation: https://openrocket.sourceforge.net/techdoc.pdf
% The spincan spins freely, so the fins transmit no roll torque to the body.
% Roll moment on the body comes from the canards only.
% Body axes: x forward (nose), y right, z down.
% Cg, CP and every X_* are measured from the NOSE TIP

%% DYNAMIC SYSTEM VARIABLES
V = max(V_raw, 0.001); % to prevent /0 errors on launchpad (V = 0)
Mach = V / a;
d = Diam; % reference length = BODY TUBE diameter (Sec. 3.1.1)
Aref = Area; % reference area = body tube area (Sec. 3.1.1)

rb = d/2; % body tube radius (nose base, tube, canards)
rs = spincan_radius; % spincan radius (fins, base)
d_sc = 2*rs; % spincan diameter
A_b = pi*rb^2; % body tube cross-section
A_s = pi*rs^2; % spincan cross-section

p_rate = omega(1);  q_rate = omega(2);  r_rate = omega(3);

K_bl = 1.1; % body-lift constant K, for Eq. 3.26

% 2 canards
% equal deflection = roll control, differential = pitch control (no yaw authority).
phi_CR = [0, pi];
N_CR = numel(phi_CR); % number of canards

% GEOMETRY 
L_rocket = Booster_Length;
x_TR = L_rocket - SC_L - 2*TR_L; % fore transition start
x_SC = x_TR + TR_L; % spincan start
x_AT = x_SC + SC_L; % aft transition start (ends at the base, radius rb)
L_tube = x_TR - NC_L; % body tube length (between nose and transition)

% total AoA & direction of the normal force
sin_at = sqrt(sin(beta)^2 + (cos(beta)*sin(alpha))^2); % sin(alpha_total)
cos_at = cos(alpha)*cos(beta);
alpha_t = atan2(sin_at, cos_at); % total AoA
alpha_c = max(alpha_t, 1e-4); % so that alpha is not 0
if sin_at > 1e-9
    e_lat = [sin(beta); cos(beta)*sin(alpha)] / sin_at;
else
    e_lat = [0; 0];
end

%% NORMAL FORCE & CENTRE OF PRESSURE  (modified Barrowman)

sa_over_a = sin(alpha_c)/alpha_c; % sin(alpha)/alpha correction from Eq. 3.19
sa2_over_a = sin(alpha_c)^2/alpha_c; % sin^2(alpha)/alpha, body lift Eq. 3.26

% Nose cone (potential-flow part)
CNa_NC = (2/Aref)*(NC_aBase - NC_aTop)*sa_over_a; % Eq. 3.19
X_NC = NC_CP; % for the ogive: 0.466*NC_L (from constants file)

% Nose cone body lift (Galejs modification)
CNa_L_NC = K_bl*(NC_aPlan/Aref)*sa2_over_a; % Eq. 3.26
X_L_NC = NC_Xlift; % Eq. 3.27 (for an ogive nosecone, calculated in constants file)

% Body tube (body lift only)
CNa_L_T = K_bl*(d*L_tube/Aref)*sa2_over_a; % Eq. 3.26, Aplan = d*l
X_L_T = NC_L + L_tube/2; % Eq. 3.27 (cylinder: mid-length)

% Conical transition body tube -> spincan (diverging, so it generates positive normal force)
CNa_TR = (2/Aref)*(A_s - A_b)*sa_over_a; % Eq. 3.19 (transition: aft area - fore area)
X_TR_CP = x_TR + (TR_L/3)*(1 + 1/(1 + rb/rs)); % Barrowman conical-transition CP
CNa_L_TR = K_bl*((TR_L*(d + d_sc)/2)/Aref)*sa2_over_a; % Eq. 3.26, Aplan = trapezoid
X_L_TR = x_TR + TR_L*(d + 2*d_sc)/(3*(d + d_sc)); % Eq. 3.27 (centroid of trapezoidal planform)

% Spincan (body lift only)
CNa_L_SC = K_bl*(d_sc*SC_L/Aref)*sa2_over_a; % Eq. 3.26, Aplan = d_sc*l
X_L_SC = x_SC + SC_L/2; % Eq. 3.27

% Aft transition spincan -> body diameter (converging, so negative normal force; nets to zero with the fore transition)
CNa_AT = (2/Aref)*(A_b - A_s)*sa_over_a; % Eq. 3.19 (aft area - fore area < 0)
X_AT_CP = x_AT + (TR_L/3)*(1 + 1/(1 + rs/rb)); % Barrowman conical-transition CP (d_fore/d_aft = rs/rb)
CNa_L_AT = K_bl*((TR_L*(d + d_sc)/2)/Aref)*sa2_over_a; % Eq. 3.26, Aplan = trapezoid
X_L_AT = x_AT + TR_L*(d_sc + 2*d)/(3*(d_sc + d)); % Eq. 3.27 (centroid of trapezoidal planform)

% Fins (mounted on the spincan, so root radius = rs)
KTB_BF = 1 + rs/(BF_H + rs); % Eq. 3.56
CN1_BF = finCN1(alpha_c, Mach, BF_H, BF_plan, Gc_BF, Aref); % Eq. 3.40 (M<0.9) / 3.48-3.49 (M>1.3)
CNa_BF = KTB_BF*finCountFactor(BF_NFins)*(BF_NFins/2)*CN1_BF/alpha_c; % Eq. 3.53, 3.54, 3.55
X_BF = BF_X + xMAC_BF + finCPfrac(Mach, BF_H, BF_plan)*cbar_BF; % Eq. 3.34 / 3.35 / 3.36

% Totals
CNa_Total = CNa_NC + CNa_L_NC + CNa_L_T + CNa_TR + CNa_L_TR + CNa_L_SC + CNa_AT + CNa_L_AT + CNa_BF;
CP_Total = (CNa_NC*X_NC + CNa_L_NC*X_L_NC + CNa_L_T*X_L_T + CNa_TR*X_TR_CP + CNa_L_TR*X_L_TR ...
          + CNa_L_SC*X_L_SC + CNa_AT*X_AT_CP + CNa_L_AT*X_L_AT + CNa_BF*X_BF) / CNa_Total; % Eq. 3.29

CN_Total = CNa_Total*alpha_t; % Eq. 3.8
N_force  = q*Aref*CN_Total; % Eq. 3.1

Fy_N = -N_force*e_lat(1); % lateral force opposes lateral airflow
Fz_N = -N_force*e_lat(2);

arm = CP_Total - Cg; % CP aft of CG => stable (Eq. 3.3 / 3.4)
My_N = Fz_N*arm; % Eq. 3.3 (moment of N about the CG)
Mz_N = -Fy_N*arm; % Eq. 3.3

%% BODY OUTLINE (used for wetted area and pitch/yaw damping)
% Tangent-ogive nose, tube, flare, spincan, taper back to tube radius. Built once.
persistent x_prof r_prof A_wet_body
if isempty(x_prof)
    Np = 400;
    x_prof = linspace(0, L_rocket, Np)';
    r_prof = bodyRadius(x_prof, NC_L, rb, x_TR, TR_L, rs, x_AT);
    A_wet_body = sum(pi*(r_prof(1:end-1) + r_prof(2:end)).*sqrt(diff(x_prof).^2 + diff(r_prof).^2));
end

%% AXIAL DRAG  CD0 = friction + nose/transition pressure + fin pressure + base
Reynolds = V*L_rocket/kinematic_visc; % Eq. 3.12
R_crit = 51*(SurfaceRoughness/L_rocket)^(-1.039); % Eq. 3.79
rough = (Reynolds >= 1e4) && (Reynolds >= R_crit);

if Reynolds < 1e4
    Cf_t = 1.48e-2; % Eq. 3.81 (R < 1e4)
    Cf   = Cf_t;
else
    Cf_t = 1/(1.50*log(Reynolds) - 5.6)^2; % Eq. 3.78
    if Reynolds < R_crit
        Cf = Cf_t; % Eq. 3.81 (1e4 < R < R_crit)
    else
        Cf = 0.032*(SurfaceRoughness/L_rocket)^0.2; % Eq. 3.80
    end
end

% compressibility correction, blended over 0.9 < M < 1.1 (no jump at M = 1)
Cf_sub = Cf*(1 - 0.1*Mach^2); % Eq. 3.82
Cf_sup = Cf_t/(1 + 0.15*Mach^2)^0.58; % Eq. 3.83
if rough
    Cf_sup = max(Cf/(1 + 0.18*Mach^2), Cf_sup); % Eq. 3.84 (not allowed below turbulent value)
end
if Mach <= 0.9
    Cf_c = Cf_sub;
elseif Mach >= 1.1
    Cf_c = Cf_sup;
else
    w_cf = (Mach - 0.9)/0.2;
    Cf_c = (1 - w_cf)*Cf_sub + w_cf*Cf_sup;
end

f_B = L_rocket/d_sc; % fineness ratio, Sec. 3.1.3 (based on the maximum diameter)
A_wet_fin = (1 + 2*BF_t/cbar_BF)*2*BF_NFins*BF_plan; % both sides, thickness-corrected (Eq. 3.85)
if CR_Plan > 0
    A_wet_fin = A_wet_fin + (1 + 2*CR_t/cbar_CR)*2*N_CR*CR_Plan; % Eq. 3.85
end
CD_fric = Cf_c*((1 + 1/(2*f_B))*A_wet_body + A_wet_fin)/Aref; % Eq. 3.85

% nose-cone pressure drag, referenced to Aref
CD_nose = (NC_aBase/Aref)*noseCD(Mach, NC_L, NC_dBase, NC_phiJoint, NC_kappa); % Eq. 3.75, 3.86, 3.87, B.3-B.8

% transition (diverging cone) pressure drag: nose-cone relations with the transition half-angle, cone shape (Fog = 1)
if rs > rb + 1e-9
    eps_TR = atan((rs - rb)/TR_L);
    CD_TR = ((A_s - A_b)/Aref)*noseCD(Mach, TR_L, d_sc - d, eps_TR, 1); % Eq. 3.75, 3.86, 3.87, B.3-B.8 (dN = 2*(rs-rb), phi = eps)
else
    CD_TR = 0;
end

% fin pressure drag (leading edge + trailing edge), referenced to Aref
CD_finp = finPresCD(Mach, BF_NFins, BF_t, BF_H, BF_SA, Aref); % Eq. 3.90-3.93, 3.75
if CR_Plan > 0
    CD_finp = CD_finp + finPresCD(Mach, N_CR, CR_t, CR_Span, CR_LE, Aref); % Eq. 3.90-3.93, 3.75
end

% base drag: the base is the end of the aft transition (body diameter), minus the thrusting motor's area (Sec. 3.4.5)
if thrust_on > 0
    A_motor = pi*(Booster_MotorDiam/2)^2;
else
    A_motor = 0;
end
A_base  = max(A_b - A_motor, 0); % base is the end of the aft transition (radius rb), not the spincan
CD_base = (A_base/Aref)*baseCD(Mach); % Eq. 3.94, Eq. 3.75

CD0 = CD_fric + CD_nose + CD_TR + CD_finp + CD_base; % Eq. 3.97
CA  = CD0*axialAoAFactor(alpha_t); % Sec. 3.4.7 (CA from CD0, 1 -> 1.3 @17deg -> 0 @90deg)

Fx_N = -q*Aref*CA; % Eq. 3.9 (axial force, drag opposes +x)

%% PITCH / YAW DAMPING  - Sec. 3.2.3
% Body: crossflow drag over the real outline, 2*Cdc*int(r(x)*|x-Cg|^3 dx) with Cdc = 1.1.
% For a constant radius this reduces to 0.55*r*(lf^4 + lr^4) of Eq. 3.59.
I_body = trapz(x_prof, r_prof.*abs(x_prof - Cg).^3);
Cdamp_unit = 2.2*I_body/(Aref*d); % Eq. 3.59 (body fore + aft of CG, local radius), per (w^2/V^2)
Cdamp_unit = Cdamp_unit + 0.6*min(BF_NFins,4)*BF_plan*abs(X_BF - Cg)^3/(Aref*d); % Eq. 3.60
if CR_Plan > 0
    Cdamp_unit = Cdamp_unit + 0.6*N_CR*CR_Plan*abs(CR_pos - Cg)^3/(Aref*d); % Eq. 3.60 (canards treated as a fin set)
end
My_D = -sign(q_rate)*q*Aref*d*Cdamp_unit*q_rate^2/V^2; % Eq. 3.59/3.60, opposite to pitch rate
Mz_D = -sign(r_rate)*q*Aref*d*Cdamp_unit*r_rate^2/V^2; % same correction applied to yaw (Sec. 3.2.3)

%% CANARDS (N_CR independently deflected fins on the BODY TUBE, radius rb) - treated as fins
Fx_c = 0;  Fy_c = 0;  Fz_c = 0;
Mx_c = 0;  My_c = 0;  Mz_c = 0;

if CR_Plan > 0
    KTB_CR = 1 + rb/(CR_Span + rb); % Eq. 3.56 (canards sit on the body tube, not the spincan)
    xi_CR = CR_yMAC + rb; % lever arm, Eq. 3.66
    arm_CR = CR_pos - Cg; % axial arm of canard lift about CG
    eta_CR = atan(p_rate*xi_CR/V); % Eq. 3.62 (roll-rate incidence at the MAC)

    for i = 1:N_CR
        s_loc = -sin(phi_CR(i))*sin(beta) + cos(phi_CR(i))*cos(beta)*sin(alpha); % Eq. 3.50 (alpha_i = alpha*sin(Lambda_i))
        a_loc = asin(max(min(s_loc, 1), -1));
        a_eff = a_loc + eta_CR - canard_angle(i); % Eq. 3.63 (sign flipped: force acts along -n_i)
        CN_i  = KTB_CR*finCN1(a_eff, Mach, CR_Span, CR_Plan, CR_mC, Aref); % Eq. 3.40 / 3.49, Eq. 3.55

        Fy_c = Fy_c + q*Aref*CN_i*sin(phi_CR(i)); % Eq. 3.1 resolved on y
        Fz_c = Fz_c - q*Aref*CN_i*cos(phi_CR(i)); % Eq. 3.1 resolved on z
        Mx_c = Mx_c - q*Aref*CN_i*xi_CR; % Eq. 3.66 (roll forcing + roll damping of the canards)
        Fx_c = Fx_c - q*Aref*abs(CN_i)*abs(sin(canard_angle(i))); % deflection (induced) drag - extension, NOT in OpenRocket
    end
    My_c =  Fz_c*arm_CR; % Eq. 3.3
    Mz_c = -Fy_c*arm_CR; % Eq. 3.3
end

%% OUTPUT ASSEMBLY
Fxyz = [Fx_N + Fx_c;
        Fy_N + Fy_c;
        Fz_N + Fz_c];

Mxyz = [Mx_c;
        My_N + My_D + My_c;
        Mz_N + Mz_D + Mz_c];
end


%% LOCAL FUNCTIONS  (to clean up the rest of the code)

function r = bodyRadius(x, L_nc, rb, x_tr, L_tr, rs, x_at)
% Outline radius vs. distance from nose tip: tangent ogive, tube, linear flare, spincan, linear taper to tube radius.
    rho = (rb^2 + L_nc^2)/(2*rb); % tangent-ogive radius of curvature
    r = rs*ones(size(x)); % spincan by default
    m1 = x < L_nc;
    m2 = (x >= L_nc) & (x < x_tr);
    m3 = (x >= x_tr) & (x < x_tr + L_tr);
    m4 = (x >= x_at);
    r(m1) = sqrt(max(rho^2 - (L_nc - x(m1)).^2, 0)) + rb - rho;
    r(m2) = rb;
    r(m3) = rb + (rs - rb)*(x(m3) - x_tr)/L_tr;
    r(m4) = rs + (rb - rs)*(x(m4) - x_at)/L_tr;
    r = max(r, 0);
end

function CN1 = finCN1(ae, M, s, Afin, Gc, Aref)
% Normal-force coefficient of ONE fin @ incidence ae
% Subsonic Diederich (M<=0.9), supersonic Busemann (M>=1.3), linear blend in between
    if M <= 0.9
        CN1 = finSub(ae, M, s, Afin, Gc, Aref);
    elseif M >= 1.3
        CN1 = finSup(ae, M, Afin, Aref);
    else
        w = (M - 0.9)/0.4;
        CN1 = (1 - w)*finSub(ae, 0.9, s, Afin, Gc, Aref) + w*finSup(ae, 1.3, Afin, Aref);
    end
end

function CN1 = finSub(ae, M, s, Afin, Gc, Aref)
    beta_c = sqrt(1 - M^2); % Eq. 3.13 (M<1)
    CNa1 = 2*pi*(s^2/Aref)/(1 + sqrt(1 + (beta_c*s^2/(Afin*cos(Gc)))^2)); % Eq. 3.40
    CN1 = CNa1*ae; % Eq. 3.7 / 3.8
end

function CN1 = finSup(ae, M, Afin, Aref)
    gam = 1.4;
    b = sqrt(M^2 - 1); % Eq. 3.13 (M>1)
    K1 = 2/b; % Eq. 3.42
    K2 = ((gam + 1)*M^4 - 4*b^2)/(4*b^4); % Eq. 3.43
    K3 = ((gam + 1)*M^8 + (2*gam^2 - 7*gam - 5)*M^6 + 10*(gam + 1)*M^4 + 8)/(6*b^7); % Eq. 3.44
    aa = abs(ae);
    CN1 = sign(ae)*(Afin/Aref)*(K1*aa + K2*aa^2 + K3*aa^3); % Eq. 3.41, 3.48, 3.49
end

function f = finCountFactor(Ntot)
% Fin-fin interference factor for many fins, Eq. 3.54
    if Ntot <= 4
        f = 1.000;
    elseif Ntot == 5
        f = 0.948;
    elseif Ntot == 6
        f = 0.913;
    elseif Ntot == 7
        f = 0.854;
    elseif Ntot == 8
        f = 0.810;
    else
        f = 0.750;
    end
end

function f = finCPfrac(M, s, Afin)
% CP position as a fraction of the MAC, measured from the MAC leading edge.
    AR = 2*s^2/Afin; % aspect ratio used by Eq. 3.35
    if M <= 0.5
        f = 0.25; % Barrowman quarter-chord (Sec. 3.2.2)
    elseif M >= 2
        b = sqrt(M^2 - 1);
        f = (AR*b - 0.67)/(2*AR*b - 1); % Eq. 3.35
    else % use 5th order polynomial approximation for graph
        b2 = sqrt(3); % beta at M = 2
        f2 = (AR*b2 - 0.67)/(2*AR*b2 - 1); % f(2), Eq. 3.35
        df2 = 0.34*AR*2/(b2*(2*AR*b2 - 1)^2); % f'(2), derivative of Eq. 3.35
        Am = [1 0.5 0.25 0.125 0.0625 0.03125;
              0 1   1    0.75  0.5    0.3125;
              1 2   4    8     16     32;
              0 1   4    12    32     80;
              0 0   2    12    48     160;
              0 0   0    6     48     240];
        rhs = [0.25; 0; f2; df2; 0; 0]; % constraints, Eq. 3.36
        c = Am\rhs;
        f = c(1) + c(2)*M + c(3)*M^2 + c(4)*M^3 + c(5)*M^4 + c(6)*M^5; % 5th-order polynomial p(M), Eq. 3.36
    end
end

function CD = noseCD(M, L, dN, phiJ, kappa)
% Nose-cone pressure-drag coefficient referenced to the nose base area (CD_bullet).
% Also used for the diverging transition: L = transition length, dN = 2*(rs - rb), phiJ = half-angle, kappa = 1.
    gam = 1.4;
    fN  = L/dN; % nose fineness ratio
    ep  = atan(1/(2*fN)); % Eq. B.3
    se  = sin(ep);
    Fog = 0.72*(kappa - 0.5)^2 + 0.82; % Eq. B.8 (ogive shape factor; 1.0 for tangent ogive)
    CDp0 = 0.8*sin(phiJ)^2; % Eq. 3.86
    CD1  = Fog*(1.0*se); % Eq. B.6  (value at M = 1)
    dCD1 = Fog*(4/(gam + 1))*(1 - 0.5*(1.0*se)); % Eq. B.5  (slope at M = 1)
    if M <= 1
        a_c = CD1 - CDp0;
        b_c = dCD1/a_c;
        CD  = a_c*M^b_c + CDp0; % Eq. 3.87 (a, b fitted to B.6 and B.5)
    elseif M >= 1.3
        CD  = Fog*(2.1*se^2 + 0.5*se/sqrt(M^2 - 1)); % Eq. B.4
    else
        M2 = 1.3;
        v2 = Fog*(2.1*se^2 + 0.5*se/sqrt(M2^2 - 1)); % Eq. B.4 at M = 1.3
        m2 = Fog*(-0.5*se*M2*(M2^2 - 1)^(-1.5)); % d/dM of Eq. B.4 at M = 1.3
        h  = M2 - 1;
        t  = (M - 1)/h;
        h00 =  2*t^3 - 3*t^2 + 1;
        h10 =  t^3 - 2*t^2 + t;
        h01 = -2*t^3 + 3*t^2;
        h11 =  t^3 - t^2;
        CD  = h00*CD1 + h10*h*dCD1 + h01*v2 + h11*h*m2; % cubic through B.4, B.5, B.6 (Sec. B.2)
    end
end

function CD = baseCD(M)
    if M < 1
        CD = 0.12 + 0.13*M^2; % Eq. 3.94
    else
        CD = 0.25/M; % Eq. 3.94
    end
end

function r = qStagRatio(M)
    if M < 1
        r = 1 + M^2/4 + M^4/40; % Eq. B.1
    else
        r = 1.84 - 0.76/M^2 + 0.166/M^4 + 0.035/M^6; % Eq. B.1
    end
end

function CD = finPresCD(M, Nf, t, s, GL, Aref)
% Fin pressure drag, rectangular (square-edged) fin profile, referenced to Aref.
    CD_stag = 0.85*qStagRatio(M); % Eq. B.2
    CD_LEp = CD_stag; % Eq. 3.90
    CD_LE = CD_LEp*cos(GL)^2; % Eq. 3.91
    CD_TE = baseCD(M); % Eq. 3.92 (square profile = body base drag, Eq. 3.94)
    CD = (Nf*t*s/Aref)*(CD_LE + CD_TE); % Eq. 3.93, scaled by Eq. 3.75 (ref. area = N*t*s)
end

function f = axialAoAFactor(at)
% CA/CD0 vs. angle of attack (Sec. 3.4.7): two cubic pieces, f(0)=1, f(17deg)=1.3, f(90deg)=0, zero slope @ all three.
    a1 = 17*pi/180;
    a2 = pi/2;
    at = min(max(at, 0), a2);
    if at <= a1
        t = at/a1;
        f = 1 + 0.3*(3*t^2 - 2*t^3);
    else
        t = (at - a1)/(a2 - a1);
        f = 1.3*(1 - (3*t^2 - 2*t^3));
    end
end
